simulink model "QAM_and_linear_equalization"  (R2024a)
settings: Solver=VariableStepAuto  StartTime=0.0  StopTime=10.0  RelTol=1e-3
undefined symbols (not defined in the file): j
libraries: commchan3 x1, commeq3 x1, commrandsrc3 x1, commdigbbndam3 x1, matrix_library x1
settings Model: Creator=Anusnekhaa Narendran  LastModifiedBy=Anusnekhaa Narendran

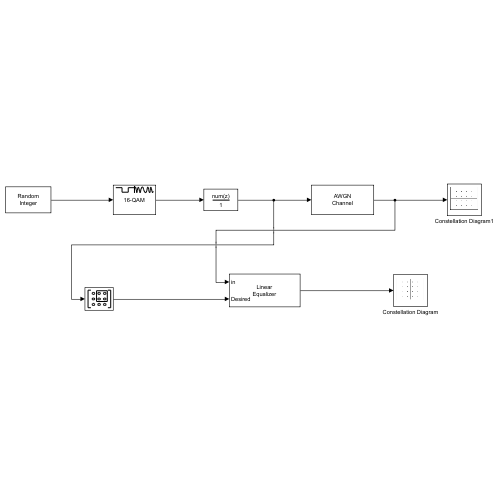
[thumbnail: Simulink's stored preview of the top-level diagram]
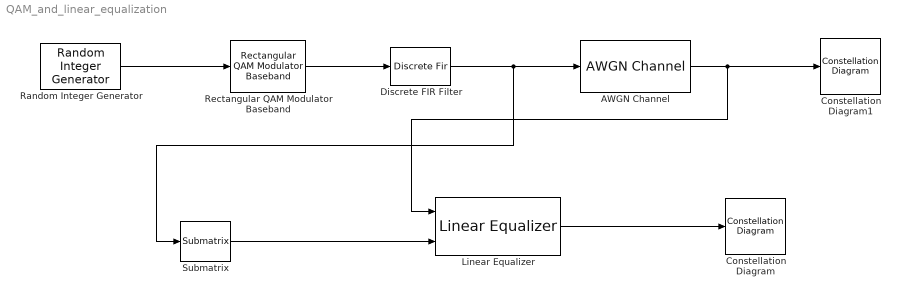
== system QAM_and_linear_equalization ==
  AWGN Channel : commchan3/AWGN Channel  LegacyMode=off  NoiseMethod="Signal to noise ratio  (Eb/No)"  noiseMode="Signal to noise ratio  (SNR)"  EbNo=40  EsNo=10  SNR=10  BitsPerSymbol=4  SignalPower=1e-3  SamplesPerSymbol=2  SymbolPeriod=1  VarianceSource=Parameter  Variance=1  RandomStream=Global stream  Seed=67  SimulateUsing=Code generation
  Constellation Diagram : ConstellationDiagram  WindowPosition=[1.000000,49.000000,1536.000000,792.000000,]  ScopeFrameLocation=window
  Constellation Diagram1 : ConstellationDiagram  WindowPosition=[382.000000,84.000000,600.000000,600.000000,]  ScopeFrameLocation=window
  Discrete FIR Filter : DiscreteFir  Coefficients=[1 -0.3 0.1 0.2]  InputProcessing=Columns as channels (frame based)
  Linear Equalizer : commeq3/Linear Equalizer  NumTaps=6  Constellation=[-3+3j -3+j -3-j -3-3j -1+3j -1+j -1-j -1-3j 1+3j 1+j 1-j 1-3j 3+3j 3+j 3-j 3-3j]  InputSamplesPerSymbol=1  Algorithm=LMS  StepSize=0.01  ForgettingFactor=0.99  InitialInverseCorrelationMatrix=0.1  ReferenceTap=2  InputDelay=0  AdaptWeightsSource=Property  AdaptWeights=on  InitialWeightsSource=Auto  InitialWeights=0  TrainingInitialWeights=0  BlindInitialWeights=[ 0; 0; 1; 0; 0 ]  WeightUpdatePeriod=1  TrainingFlagInputPort=off  AdaptAfterTraining=on  ResetInputPort=off  ErrorOutputPort=off  TapWeightsOutputPort=off  SimulateUsing=Code generation
  Random Integer Generator : commrandsrc3/Random Integer Generator  SetSize=16  SeedSource=Auto  Seed=0  SampleTime=1e-6  SamplesPerFrame=1000  OutputDataType=double  SimulateUsing=Interpreted execution
  Rectangular QAM Modulator Baseband : commdigbbndam3/Rectangular QAM Modulator Baseband  M=16  InType=Integer  Enc=Gray  Mapping=[0:15]  PowType=Min. distance between symbols  MinDist=2  AvgPow=1  PeakPow=1  Ph=0  outDtype=double  outWordLen=16  outUDDataType=sfix(16)  outFracLenMode=Best precision  outFracLen=15  outDataTypeStr=double  outLastDataTypeStr=double
  Submatrix : matrix_library/Submatrix  RowSpan=Range of rows  RowStartMode=Index  RowStartIndex=1  RowEndMode=Index  RowEndIndex=100  ColSpan=One column  ColStartMode=First  ColStartIndex=1  ColEndMode=Last  ColEndIndex=1
  wires:
  Random Integer Generator/1 -> Rectangular QAM Modulator Baseband/1
  Rectangular QAM Modulator Baseband/1 -> Discrete FIR Filter/1
  Discrete FIR Filter/1 -> Submatrix/1, AWGN Channel/1
  AWGN Channel/1 -> Linear Equalizer/1, Constellation Diagram1/1
  Submatrix/1 -> Linear Equalizer/2
  Linear Equalizer/1 -> Constellation Diagram/1
